simulink model "L2_Sim_QPSK_2"  (R2023b)
settings: Solver=VariableStepAuto  StartTime=0.0  StopTime=100000  RelTol=1e-3
libraries: commdigbbndpm3 x4, commchan3 x2, commsink2 x2, commrflib2 x1, commrandsrc2 x1
settings Model: Creator=Liu  LastModifiedBy=Liu

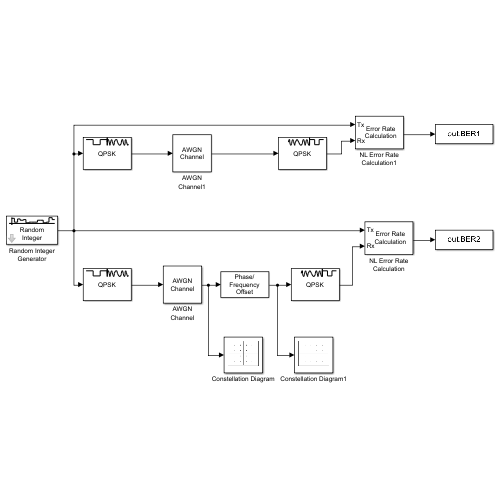
[thumbnail: Simulink's stored preview of the top-level diagram]
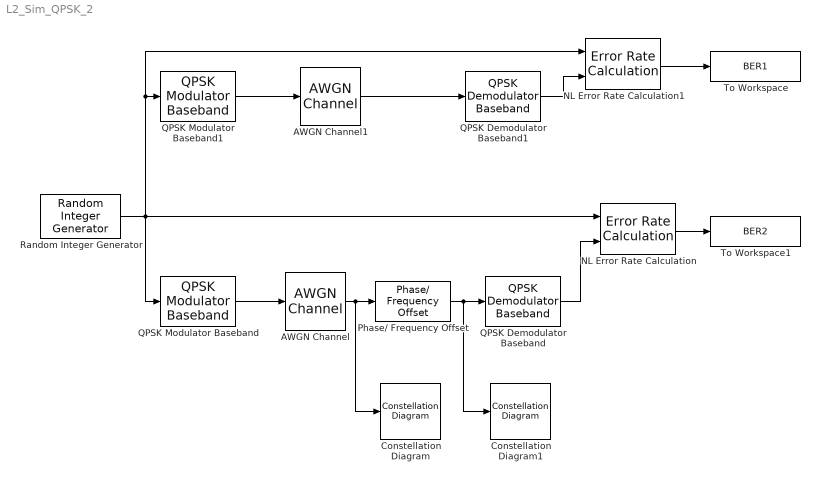
== system L2_Sim_QPSK_2 ==
  AWGN Channel : commchan3/AWGN Channel  LegacyMode=on  NoiseMethod="Signal to noise ratio  (SNR)"  noiseMode="Signal to noise ratio  (Eb/No)"  EbNo=10  EsNo=10  SNR=10  BitsPerSymbol=1  SignalPower=1  SamplesPerSymbol=1  SymbolPeriod=1  VarianceSource=Parameter  Variance=1  RandomStream=Global stream  Seed=67  SimulateUsing=Code generation
  AWGN Channel1 : commchan3/AWGN Channel  LegacyMode=on  NoiseMethod="Signal to noise ratio  (SNR)"  noiseMode="Signal to noise ratio  (Eb/No)"  EbNo=10  EsNo=10  SNR=10  BitsPerSymbol=1  SignalPower=1  SamplesPerSymbol=1  SymbolPeriod=1  VarianceSource=Parameter  Variance=1  RandomStream=Global stream  Seed=67  SimulateUsing=Code generation
  Constellation Diagram : ConstellationDiagram  WindowPosition=[382.000000,84.000000,600.000000,600.000000,]  ScopeFrameLocation=window  SymbolsToDisplaySource=Property  SymbolsToDisplay=10000  XLimits=[-1.46,1.46]  YLimits=[-1.38,1.38]
  Constellation Diagram1 : ConstellationDiagram  WindowPosition=[1.000000,49.000000,1707.000000,889.000000,]  ScopeFrameLocation=window  SymbolsToDisplaySource=Property  SymbolsToDisplay=10000  XLimits=[-1.46,1.46]  YLimits=[-1.38,1.38]
  NL Error Rate Calculation : commsink2/Error Rate Calculation  N=0  st_delay=0  cp_mode=Entire frame  subframe=[]  PMode=Port  WsName=ErrorVec  RsMode2=off  stop=off  numErr=100  maxBits=1e6
  NL Error Rate Calculation1 : commsink2/Error Rate Calculation  N=0  st_delay=0  cp_mode=Entire frame  subframe=[]  PMode=Port  WsName=ErrorVec  RsMode2=off  stop=off  numErr=100  maxBits=1e6
  Phase/ Frequency Offset : commrflib2/Phase// Frequency Offset  phaseOffset=25  freqPort=off  freqOffset=0
  QPSK Demodulator Baseband : commdigbbndpm3/QPSK Demodulator Baseband  OutType=Integer  DecType=Hard decision  VarSource=Dialog  Variance=1  Dec=Gray  Ph=pi/4  outDtype1=Inherit via internal rule  outDtype2=Inherit via internal rule  derotateFactorWordLen=16  derotateFactorDataTypeStr=Inherit: Same word length as input  derotateFactorLastDataTypeStr=Inherit: Same word length as input
  QPSK Demodulator Baseband1 : commdigbbndpm3/QPSK Demodulator Baseband  OutType=Integer  DecType=Hard decision  VarSource=Dialog  Variance=1  Dec=Gray  Ph=pi/4  outDtype1=Inherit via internal rule  outDtype2=Inherit via internal rule  derotateFactorWordLen=16  derotateFactorDataTypeStr=Inherit: Same word length as input  derotateFactorLastDataTypeStr=Inherit: Same word length as input
  QPSK Modulator Baseband : commdigbbndpm3/QPSK Modulator Baseband  InType=Integer  Enc=Gray  Ph=pi/4  outDtype=double  outWordLen=16  outUDDataType=sfix(16)  outFracLenMode=Best precision  outFracLen=15  outDataTypeStr=double  outLastDataTypeStr=double
  QPSK Modulator Baseband1 : commdigbbndpm3/QPSK Modulator Baseband  InType=Integer  Enc=Gray  Ph=pi/4  outDtype=double  outWordLen=16  outUDDataType=sfix(16)  outFracLenMode=Best precision  outFracLen=15  outDataTypeStr=double  outLastDataTypeStr=double
  Random Integer Generator : commrandsrc2/Random Integer Generator  mul=4  seed=37  Ts=1  frameBased=off  sampPerFrame=1000  orient=off  outDataType=double
  To Workspace : ToWorkspace  VariableName=BER1  SaveFormat=Timeseries  SampleTime=-1
  To Workspace1 : ToWorkspace  VariableName=BER2  SaveFormat=Timeseries  SampleTime=-1
  wires:
  AWGN Channel/1 -> Constellation Diagram/1, Phase/ Frequency Offset/1
  QPSK Demodulator Baseband/1 -> NL Error Rate Calculation/2
  Random Integer Generator/1 -> NL Error Rate Calculation1/1, QPSK Modulator Baseband1/1, NL Error Rate Calculation/1, QPSK Modulator Baseband/1
  QPSK Modulator Baseband/1 -> AWGN Channel/1
  QPSK Modulator Baseband1/1 -> AWGN Channel1/1
  AWGN Channel1/1 -> QPSK Demodulator Baseband1/1
  QPSK Demodulator Baseband1/1 -> NL Error Rate Calculation1/2
  Phase/ Frequency Offset/1 -> Constellation Diagram1/1, QPSK Demodulator Baseband/1
  NL Error Rate Calculation1/1 -> To Workspace/1
  NL Error Rate Calculation/1 -> To Workspace1/1
